simulink model "drive_brake"  (R2026b)
settings: Solver=VariableStepAuto
undefined symbols (not defined in the file or in its folder): P
libraries: nesl_utility x2, fl_lib x1
settings Model: Creator=aomar  LastModifiedBy=aomar

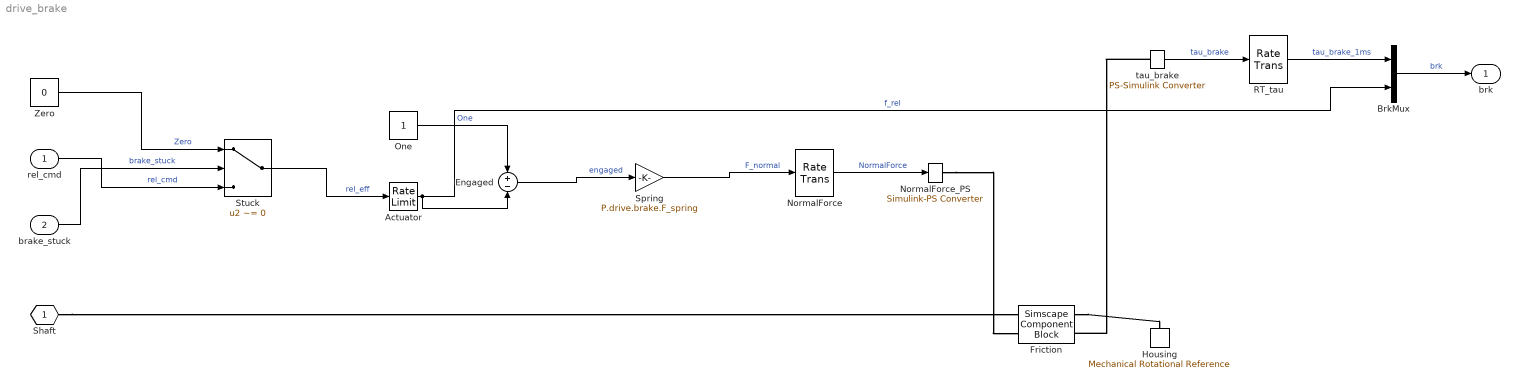
== system drive_brake ==
  rel_cmd : Inport  OutDataTypeStr=double  SampleTime=P.drive.Ts_esc
  brake_stuck : Inport  Port=2  OutDataTypeStr=boolean  SampleTime=P.drive.Ts_esc
  Actuator : RateLimiter  RisingSlewLimit=1/P.drive.brake.t_release  FallingSlewLimit=-1/P.drive.brake.t_engage  SampleTimeMode=inherited
  BrkMux : Mux  Inputs=2
  Engaged : Sum  Inputs=+-
  Friction : SimscapeComponentBlock  SourceFile=shaddad_drive.elastoplastic_brake  ComponentPath=shaddad_drive.elastoplastic_brake  ComponentVariants="[\"shaddad_drive.elastoplastic_brake\"]"  ComponentVariantNames="[\"elastoplastic_brake\"]"  ClassName=elastoplastic_brake  SchemaVersion=1  r_eff=P.drive.brake.r_eff m  mu_s=P.drive.brake.mu_s  mu_c=P.drive.brake.mu_c  w_st=P.drive.brake.w_st rad/s  k_b=P.drive.brake.k_b N*m/rad  c_b=P.drive.brake.c_b N*m*s/rad  w_d=P.drive.brake.w_d rad/s  T_eps=P.drive.brake.T_eps N*m  w_eps=P.drive.brake.w_eps rad/s  w_r=P.drive.brake.w_r rad/s  N_eps=P.drive.brake.N_eps N  t_specify=off  t_priority=None  t=0 N*m  t_nominal_specify=off  t_nominal_value=1  t_nominal_unit=N*m  w_rel_specify=off  w_rel_priority=None  w_rel=0 rad/s  w_rel_nominal_specify=off  w_rel_nominal_value=1  w_rel_nominal_unit=rad/s  z_specify=off  z_priority=High  z=0 rad  z_nominal_specify=off  z_nominal_value=1  z_nominal_unit=rad
      settings: CopyFcn=simscape.sscblock.internal.componentBlockCallback(gcbh,'COPY')  PreCopyFcn=simscape.sscblock.internal.componentBlockCallback(gcbh,'PRECOPY')  PreDeleteFcn=simscape.sscblock.internal.componentBlockCallback(gcbh,'PREDELETE')
      mask Type: Elasto-Plastic Brake
  Housing : fl_lib/Mechanical/Rotational Elements/Mechanical Rotational Reference
  NormalForce : RateTransition  OutPortSampleTimeOpt=Inherit
  NormalForce_PS : nesl_utility/Simulink-PS Converter  PhysicalDomain=network_engine_domain  SubClassName=ps_input  LeftPortType=input  RightPortType=output  PseudoPeriodic=off  Frequencies=[]  NoiseDistribution=none  NoiseParameters=[]  Unit=N  AffineConversion=off  FilteringAndDerivatives=zero  SimscapeFilterOrder=1  InputFilterTimeConstant=0.001  UdotUserProvided=0
  One : Constant
  RT_tau : RateTransition  OutPortSampleTime=P.drive.Ts_esc
  Spring : Gain  Gain=P.drive.brake.F_spring
  Stuck : Switch  Criteria=u2 ~= 0  SaturateOnIntegerOverflow=off  InputSameDT=off
  Zero : Constant  Value=0
  tau_brake : nesl_utility/PS-Simulink Converter  PhysicalDomain=network_engine_domain  SubClassName=ps_output  LeftPortType=input  RightPortType=output  PseudoPeriodic=off  Frequencies=[]  VectorFormat=inherit  Unit=N*m  AffineConversion=off
  Shaft : PMIOPort  Side=Left  ConnectionType=Connection: foundation.mechanical.rotational.rotational
  brk : Outport  OutDataTypeStr=double
  wires:
  Zero/1 -> Stuck/1  "Zero"
  rel_cmd/1 -> Stuck/3  "rel_cmd"
  brake_stuck/1 -> Stuck/2  "brake_stuck"
  Stuck/1 -> Actuator/1  "rel_eff"
  One/1 -> Engaged/1  "One"
  Actuator/1 -> BrkMux/2, Engaged/2  "f_rel"
  Engaged/1 -> Spring/1  "engaged"
  Spring/1 -> NormalForce/1  "F_normal"
  NormalForce/1 -> NormalForce_PS/1  "NormalForce"
  tau_brake/1 -> RT_tau/1  "tau_brake"
  RT_tau/1 -> BrkMux/1  "tau_brake_1ms"
  BrkMux/1 -> brk/1  "brk"
  connections:
  Shaft/RConn1 -- Friction/LConn1
  NormalForce_PS/RConn1 -- Friction/LConn2
  Friction/RConn1 -- Housing/LConn1
  tau_brake/LConn1 -- Friction/RConn2
